simulink library "Vehicle_Outputs"  (R2025a)
settings: Solver=VariableStepAuto  StartTime=0.0  StopTime=10.0  RelTol=1e-3
libraries: $bdroot x30, Body_Utilities x12, sm_lib x4, nesl_utility x2
Description:
  | Simscape Vehicle Templates Library
  | 
  | Copyright 2018-2026 The MathWorks, Inc.
settings Model: Creator=smiller  LastModifiedBy=smiller
settings OptimizationCC: ReuseModelBlockBuffer=off
settings ModelReferenceCC: EnableRefExpFcnMdlSchedulingChecks=on
settings RTWCC: GPUComputeCapability=3.5

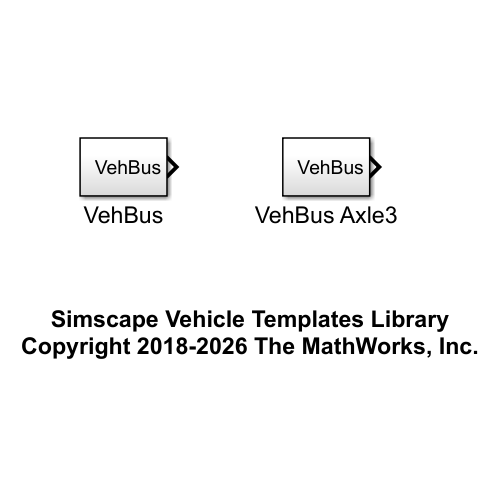
[thumbnail: Simulink's stored preview of the top-level diagram]
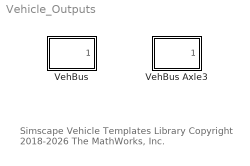
== system Vehicle_Outputs ==
  note: Simscape Vehicle Templates Library
      | Copyright 2018-2026 The MathWorks, Inc.
  VehBus : Subsystem
  VehBus Axle3 : Subsystem

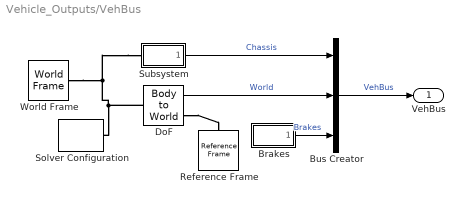
== system Vehicle_Outputs/VehBus ==
  Brakes : Subsystem
  Bus Creator : BusCreator  Inputs=3
  DoF : Body_Utilities/Body to World  VariantControl=Choice  LabelModeActiveChoice=Free  popup_BodyToWorld=Free  SpecifyPosTarget=on
  Reference Frame : sm_lib/Frames and Transforms/Reference Frame
  Solver Configuration : nesl_utility/Solver Configuration  PhysicalDomain=network_engine_domain  SubClassName=solver  LeftPortType=input  RightPortType=generic  Tones=[]  Harmonics=[]  SimulateNoise=off  Profile=off  UseLocalSampling=off  EnableSwitchedLinearOptims=on  FrequencyDomain=off  UseCCode=off  RelTol=0.001  AbsTol=1e-06  MinStep=1e-09  ToWorkspace=off  RevertToSquareIcSolve=off  NumHomotopyIterations=100  PhasorMode=off  PhasorModeNumHarmonics=1  ConsistencySolver=NEWTON_FTOL  IndexReductionMethod=DerivativeReplacement  DoDC=off  ResidualTolerance=1e-09  ConsistencyTolSource=GLOBAL  ConsistencyAbsTol=0.001  ConsistencyRelTol=0.001  ConsistencyTolFactor=0.001  UseLocalSolver=off  LocalSolverChoice=NE_BACKWARD_EULER_ADVANCER  ResolveIndetEquations=on  FunctionEvalNumThread=1  LocalSolverSampleTime=0.001  DoFixedCost=off  MaxNonlinIter=3  MaxModeIter=2  ComputeImpulses=off  ImpulseIterations=2  LinearAlgebra=auto  LinearAlgebraNumThread=0  EquationFormulation=NE_TIME_EF  DelaysMemoryBudget=1024  AutomaticFiltering=on  FilteringTimeConstant=0.001  PartitionStorageMethod=AS_NEEDED  PartitionMemoryBudget=1024  PartitionMethod=FAST  MultibodyUseLocalSolver=off  MultibodyLocalSolverChoice=ODE1  MultibodyLocalSolverSampleTime=0.001
  Subsystem : Subsystem
  World Frame : sm_lib/Frames and Transforms/World Frame
  VehBus : Outport  VectorParamsAs1DForOutWhenUnconnected=off
  wires:
  Bus Creator/1 -> VehBus/1  "VehBus"
  Subsystem/1(Chassis) -> Bus Creator/1  "Chassis"
  DoF/1 -> Bus Creator/2  "World"
  Brakes/1(Brakes) -> Bus Creator/3  "Brakes"
  connections:
  DoF/RConn1 -- Reference Frame/RConn1
  Subsystem/LConn1 -- Solver Configuration/RConn1 -- DoF/LConn1 -- World Frame/RConn1

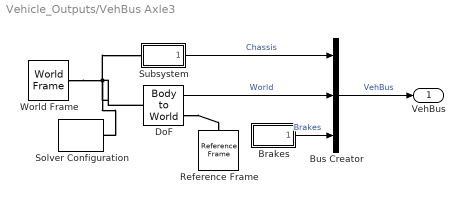
== system Vehicle_Outputs/VehBus Axle3 ==
  Brakes : Subsystem
  Bus Creator : BusCreator  Inputs=3
  DoF : Body_Utilities/Body to World  VariantControl=Choice  LabelModeActiveChoice=Free  popup_BodyToWorld=Free  SpecifyPosTarget=on
  Reference Frame : sm_lib/Frames and Transforms/Reference Frame
  Solver Configuration : nesl_utility/Solver Configuration  PhysicalDomain=network_engine_domain  SubClassName=solver  LeftPortType=input  RightPortType=generic  Tones=[]  Harmonics=[]  SimulateNoise=off  Profile=off  UseLocalSampling=off  EnableSwitchedLinearOptims=on  FrequencyDomain=off  UseCCode=off  RelTol=0.001  AbsTol=1e-06  MinStep=1e-09  ToWorkspace=off  RevertToSquareIcSolve=off  NumHomotopyIterations=100  PhasorMode=off  PhasorModeNumHarmonics=1  ConsistencySolver=NEWTON_FTOL  IndexReductionMethod=DerivativeReplacement  DoDC=off  ResidualTolerance=1e-09  ConsistencyTolSource=GLOBAL  ConsistencyAbsTol=0.001  ConsistencyRelTol=0.001  ConsistencyTolFactor=0.001  UseLocalSolver=off  LocalSolverChoice=NE_BACKWARD_EULER_ADVANCER  ResolveIndetEquations=on  FunctionEvalNumThread=1  LocalSolverSampleTime=0.001  DoFixedCost=off  MaxNonlinIter=3  MaxModeIter=2  ComputeImpulses=off  ImpulseIterations=2  LinearAlgebra=auto  LinearAlgebraNumThread=0  EquationFormulation=NE_TIME_EF  DelaysMemoryBudget=1024  AutomaticFiltering=on  FilteringTimeConstant=0.001  PartitionStorageMethod=AS_NEEDED  PartitionMemoryBudget=1024  PartitionMethod=FAST  MultibodyUseLocalSolver=off  MultibodyLocalSolverChoice=ODE1  MultibodyLocalSolverSampleTime=0.001
  Subsystem : Subsystem
  World Frame : sm_lib/Frames and Transforms/World Frame
  VehBus : Outport  VectorParamsAs1DForOutWhenUnconnected=off
  wires:
  Brakes/1(Brakes) -> Bus Creator/3  "Brakes"
  DoF/1 -> Bus Creator/2  "World"
  Subsystem/1(Chassis) -> Bus Creator/1  "Chassis"
  Bus Creator/1 -> VehBus/1  "VehBus"
  connections:
  World Frame/RConn1 -- DoF/LConn1 -- Solver Configuration/RConn1 -- Subsystem/LConn1
  DoF/RConn1 -- Reference Frame/RConn1

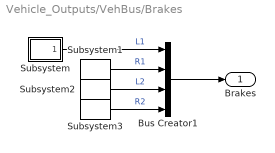
== system Vehicle_Outputs/VehBus/Brakes ==
  Bus Creator1 : BusCreator  Inputs=4
  Subsystem : Subsystem
  Subsystem1 : $bdroot/VehBus/Brakes/Subsystem  SystemSampleTime=-1  VariantActivationTime=update diagram  EmptyChoice=off  PassThrough=off  PassThroughVariantControl=(default)  EmptyChoiceVariantControl=(default)  AllowFlexibleInterface=on  Latency=0  AutoFrameSizeCalculation=off
  Subsystem2 : $bdroot/VehBus/Brakes/Subsystem  SystemSampleTime=-1  VariantActivationTime=update diagram  EmptyChoice=off  PassThrough=off  PassThroughVariantControl=(default)  EmptyChoiceVariantControl=(default)  AllowFlexibleInterface=on  Latency=0  AutoFrameSizeCalculation=off
  Subsystem3 : $bdroot/VehBus/Brakes/Subsystem  SystemSampleTime=-1  VariantActivationTime=update diagram  EmptyChoice=off  PassThrough=off  PassThroughVariantControl=(default)  EmptyChoiceVariantControl=(default)  AllowFlexibleInterface=on  Latency=0  AutoFrameSizeCalculation=off
  Brakes : Outport  VectorParamsAs1DForOutWhenUnconnected=off
  wires:
  Subsystem3/1 -> Bus Creator1/4  "R2"
  Subsystem2/1 -> Bus Creator1/3  "L2"
  Subsystem1/1 -> Bus Creator1/2  "R1"
  Subsystem/1(Whl) -> Bus Creator1/1  "L1"
  Bus Creator1/1 -> Brakes/1

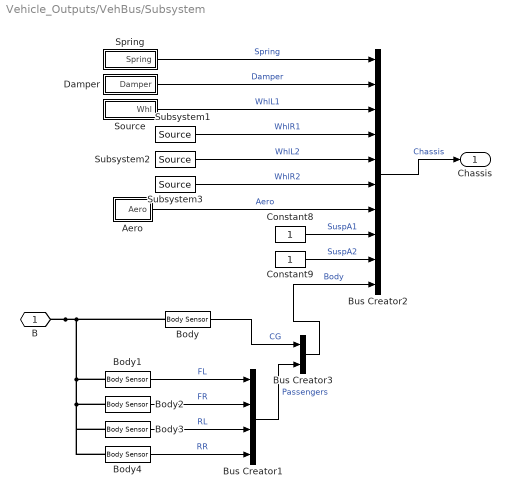
== system Vehicle_Outputs/VehBus/Subsystem ==
  Aero : Subsystem
  Body{,1..4} (5 alike) : Body_Utilities/Body Sensor  offset_body_sensor=Vehicle.Chassis.Body.sCG.Value
  Bus Creator1 : BusCreator  Inputs=4
  Bus Creator2 : BusCreator  Inputs=10
  Bus Creator3 : BusCreator  Inputs=2
  Constant8 : Constant
  Constant9 : Constant
  Damper : Subsystem
  Source : Subsystem
  Spring : Subsystem
  Subsystem1 : $bdroot/VehBus/Subsystem/Source  SystemSampleTime=-1  VariantActivationTime=update diagram  EmptyChoice=off  PassThrough=off  PassThroughVariantControl=(default)  EmptyChoiceVariantControl=(default)  AllowFlexibleInterface=on  Latency=0  AutoFrameSizeCalculation=off
  Subsystem2 : $bdroot/VehBus/Subsystem/Source  SystemSampleTime=-1  VariantActivationTime=update diagram  EmptyChoice=off  PassThrough=off  PassThroughVariantControl=(default)  EmptyChoiceVariantControl=(default)  AllowFlexibleInterface=on  Latency=0  AutoFrameSizeCalculation=off
  Subsystem3 : $bdroot/VehBus/Subsystem/Source  SystemSampleTime=-1  VariantActivationTime=update diagram  EmptyChoice=off  PassThrough=off  PassThroughVariantControl=(default)  EmptyChoiceVariantControl=(default)  AllowFlexibleInterface=on  Latency=0  AutoFrameSizeCalculation=off
  B : PMIOPort  Side=Left
  Chassis : Outport  VectorParamsAs1DForOutWhenUnconnected=off
  wires:
  Bus Creator1/1 -> Bus Creator3/2  "Passengers"
  Body4/1 -> Bus Creator1/4  "RR"
  Body3/1 -> Bus Creator1/3  "RL"
  Body2/1 -> Bus Creator1/2  "FR"
  Body1/1 -> Bus Creator1/1  "FL"
  Body/1 -> Bus Creator3/1  "CG"
  Bus Creator3/1 -> Bus Creator2/10  "Body"
  Aero/1(Aero) -> Bus Creator2/7  "Aero"
  Spring/1(Spring) -> Bus Creator2/1  "Spring"
  Source/1(Whl) -> Bus Creator2/3  "WhlL1"
  Constant9/1 -> Bus Creator2/9  "SuspA2"
  Constant8/1 -> Bus Creator2/8  "SuspA1"
  Subsystem3/1 -> Bus Creator2/6  "WhlR2"
  Subsystem2/1 -> Bus Creator2/5  "WhlL2"
  Bus Creator2/1 -> Chassis/1  "Chassis"
  Damper/1(Damper) -> Bus Creator2/2  "Damper"
  Subsystem1/1 -> Bus Creator2/4  "WhlR1"
  connections:
  B/RConn1 -- Body1/LConn1 -- Body2/LConn1 -- Body3/LConn1 -- Body4/LConn1 -- Body/LConn1

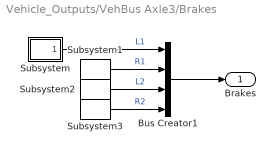
== system Vehicle_Outputs/VehBus Axle3/Brakes ==
  Bus Creator1 : BusCreator  Inputs=4
  Subsystem : Subsystem
  Subsystem1 : $bdroot/VehBus/Brakes/Subsystem  SystemSampleTime=-1  VariantActivationTime=update diagram  EmptyChoice=off  PassThrough=off  PassThroughVariantControl=(default)  EmptyChoiceVariantControl=(default)  AllowFlexibleInterface=on  Latency=0  AutoFrameSizeCalculation=off
  Subsystem2 : $bdroot/VehBus/Brakes/Subsystem  SystemSampleTime=-1  VariantActivationTime=update diagram  EmptyChoice=off  PassThrough=off  PassThroughVariantControl=(default)  EmptyChoiceVariantControl=(default)  AllowFlexibleInterface=on  Latency=0  AutoFrameSizeCalculation=off
  Subsystem3 : $bdroot/VehBus/Brakes/Subsystem  SystemSampleTime=-1  VariantActivationTime=update diagram  EmptyChoice=off  PassThrough=off  PassThroughVariantControl=(default)  EmptyChoiceVariantControl=(default)  AllowFlexibleInterface=on  Latency=0  AutoFrameSizeCalculation=off
  Brakes : Outport  VectorParamsAs1DForOutWhenUnconnected=off
  wires:
  Bus Creator1/1 -> Brakes/1
  Subsystem/1(Whl) -> Bus Creator1/1  "L1"
  Subsystem1/1 -> Bus Creator1/2  "R1"
  Subsystem2/1 -> Bus Creator1/3  "L2"
  Subsystem3/1 -> Bus Creator1/4  "R2"

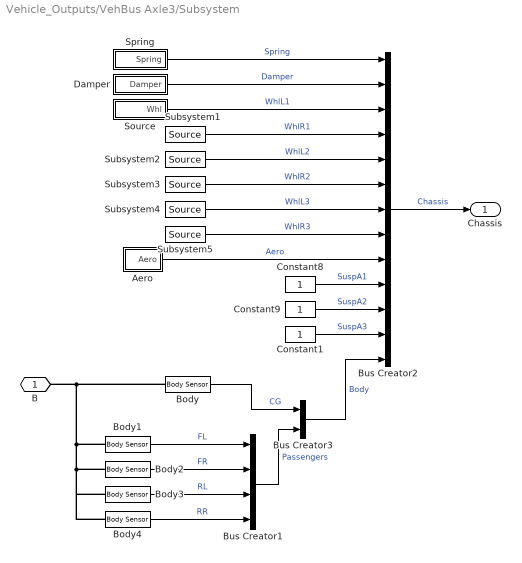
== system Vehicle_Outputs/VehBus Axle3/Subsystem ==
  Aero : Subsystem
  Body{,1..4} (5 alike) : Body_Utilities/Body Sensor  offset_body_sensor=Vehicle.Chassis.Body.sCG.Value
  Bus Creator1 : BusCreator  Inputs=4
  Bus Creator2 : BusCreator  Inputs=13
  Bus Creator3 : BusCreator  Inputs=2
  Constant1 : Constant
  Constant8 : Constant
  Constant9 : Constant
  Damper : Subsystem
  Source : Subsystem
  Spring : Subsystem
  Subsystem{1..5} (5 alike) : $bdroot/VehBus/Subsystem/Source  SystemSampleTime=-1  VariantActivationTime=update diagram  EmptyChoice=off  PassThrough=off  PassThroughVariantControl=(default)  EmptyChoiceVariantControl=(default)  AllowFlexibleInterface=on  Latency=0  AutoFrameSizeCalculation=off
  B : PMIOPort  Side=Left
  Chassis : Outport  VectorParamsAs1DForOutWhenUnconnected=off
  wires:
  Subsystem1/1 -> Bus Creator2/4  "WhlR1"
  Damper/1(Damper) -> Bus Creator2/2  "Damper"
  Bus Creator2/1 -> Chassis/1  "Chassis"
  Subsystem2/1 -> Bus Creator2/5  "WhlL2"
  Subsystem3/1 -> Bus Creator2/6  "WhlR2"
  Constant8/1 -> Bus Creator2/10  "SuspA1"
  Constant9/1 -> Bus Creator2/11  "SuspA2"
  Source/1(Whl) -> Bus Creator2/3  "WhlL1"
  Spring/1(Spring) -> Bus Creator2/1  "Spring"
  Aero/1(Aero) -> Bus Creator2/9  "Aero"
  Bus Creator3/1 -> Bus Creator2/13  "Body"
  Body/1 -> Bus Creator3/1  "CG"
  Body1/1 -> Bus Creator1/1  "FL"
  Body2/1 -> Bus Creator1/2  "FR"
  Body3/1 -> Bus Creator1/3  "RL"
  Body4/1 -> Bus Creator1/4  "RR"
  Bus Creator1/1 -> Bus Creator3/2  "Passengers"
  Subsystem5/1 -> Bus Creator2/8  "WhlR3"
  Subsystem4/1 -> Bus Creator2/7  "WhlL3"
  Constant1/1 -> Bus Creator2/12  "SuspA3"
  connections:
  Body/LConn1 -- Body4/LConn1 -- Body3/LConn1 -- Body2/LConn1 -- Body1/LConn1 -- B/RConn1

== system Vehicle_Outputs/VehBus/Brakes/Subsystem ==
  Bus Creator : BusCreator  Inputs=2
  Constant : Constant
  Constant1 : Constant
  Whl : Outport  VectorParamsAs1DForOutWhenUnconnected=off
  wires:
  Constant1/1 -> Bus Creator/2  "p"
  Bus Creator/1 -> Whl/1
  Constant/1 -> Bus Creator/1  "trq"

== system Vehicle_Outputs/VehBus/Subsystem/Aero ==
  Bus Creator : BusCreator  Inputs=2
  Constant1 : Constant
  Constant3 : Constant
  Aero : Outport  VectorParamsAs1DForOutWhenUnconnected=off
  wires:
  Bus Creator/1 -> Aero/1  "Aero"
  Constant1/1 -> Bus Creator/2  "Fz"
  Constant3/1 -> Bus Creator/1  "Fx"

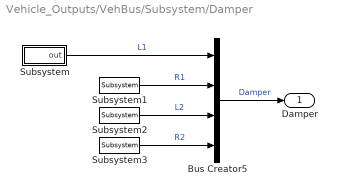
== system Vehicle_Outputs/VehBus/Subsystem/Damper ==
  Bus Creator5 : BusCreator  Inputs=4
  Subsystem : Subsystem
  Subsystem1 : $bdroot/VehBus/Subsystem/Damper/Subsystem  SystemSampleTime=-1  VariantActivationTime=update diagram  EmptyChoice=off  PassThrough=off  PassThroughVariantControl=(default)  EmptyChoiceVariantControl=(default)  AllowFlexibleInterface=on  Latency=0  AutoFrameSizeCalculation=off
  Subsystem2 : $bdroot/VehBus/Subsystem/Damper/Subsystem  SystemSampleTime=-1  VariantActivationTime=update diagram  EmptyChoice=off  PassThrough=off  PassThroughVariantControl=(default)  EmptyChoiceVariantControl=(default)  AllowFlexibleInterface=on  Latency=0  AutoFrameSizeCalculation=off
  Subsystem3 : $bdroot/VehBus/Subsystem/Damper/Subsystem  SystemSampleTime=-1  VariantActivationTime=update diagram  EmptyChoice=off  PassThrough=off  PassThroughVariantControl=(default)  EmptyChoiceVariantControl=(default)  AllowFlexibleInterface=on  Latency=0  AutoFrameSizeCalculation=off
  Damper : Outport  VectorParamsAs1DForOutWhenUnconnected=off
  wires:
  Subsystem/1(out) -> Bus Creator5/1  "L1"
  Subsystem2/1 -> Bus Creator5/3  "L2"
  Bus Creator5/1 -> Damper/1  "Damper"
  Subsystem1/1 -> Bus Creator5/2  "R1"
  Subsystem3/1 -> Bus Creator5/4  "R2"

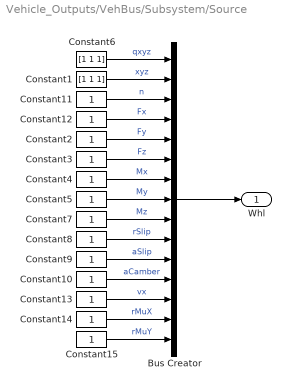
== system Vehicle_Outputs/VehBus/Subsystem/Source ==
  Bus Creator : BusCreator  Inputs=15
  Constant1 : Constant  Value=[1 1 1]
  Constant{2..5,7..15} (13 alike) : Constant
  Constant6 : Constant  Value=[1 1 1]
  Whl : Outport  VectorParamsAs1DForOutWhenUnconnected=off
  wires:
  Constant15/1 -> Bus Creator/15  "rMuY"
  Constant14/1 -> Bus Creator/14  "rMuX"
  Constant13/1 -> Bus Creator/13  "vx"
  Constant10/1 -> Bus Creator/12  "aCamber"
  Constant9/1 -> Bus Creator/11  "aSlip"
  Constant8/1 -> Bus Creator/10  "rSlip"
  Constant7/1 -> Bus Creator/9  "Mz"
  Constant5/1 -> Bus Creator/8  "My"
  Constant4/1 -> Bus Creator/7  "Mx"
  Constant3/1 -> Bus Creator/6  "Fz"
  Constant2/1 -> Bus Creator/5  "Fy"
  Bus Creator/1 -> Whl/1
  Constant6/1 -> Bus Creator/1  "qxyz"
  Constant1/1 -> Bus Creator/2  "xyz"
  Constant12/1 -> Bus Creator/4  "Fx"
  Constant11/1 -> Bus Creator/3  "n"

== system Vehicle_Outputs/VehBus/Subsystem/Spring ==
  Bus Creator5 : BusCreator  Inputs=4
  Source : Subsystem
  Source1 : $bdroot/VehBus/Subsystem/Spring/Source  SystemSampleTime=-1  VariantActivationTime=update diagram  EmptyChoice=off  PassThrough=off  PassThroughVariantControl=(default)  EmptyChoiceVariantControl=(default)  AllowFlexibleInterface=on  Latency=0  AutoFrameSizeCalculation=off
  Source2 : $bdroot/VehBus/Subsystem/Spring/Source  SystemSampleTime=-1  VariantActivationTime=update diagram  EmptyChoice=off  PassThrough=off  PassThroughVariantControl=(default)  EmptyChoiceVariantControl=(default)  AllowFlexibleInterface=on  Latency=0  AutoFrameSizeCalculation=off
  Source3 : $bdroot/VehBus/Subsystem/Spring/Source  SystemSampleTime=-1  VariantActivationTime=update diagram  EmptyChoice=off  PassThrough=off  PassThroughVariantControl=(default)  EmptyChoiceVariantControl=(default)  AllowFlexibleInterface=on  Latency=0  AutoFrameSizeCalculation=off
  Spring : Outport  VectorParamsAs1DForOutWhenUnconnected=off
  wires:
  Source/1(out) -> Bus Creator5/1  "L1"
  Source3/1 -> Bus Creator5/4  "R2"
  Source2/1 -> Bus Creator5/3  "L2"
  Source1/1 -> Bus Creator5/2  "R1"
  Bus Creator5/1 -> Spring/1  "Spring"

== system Vehicle_Outputs/VehBus Axle3/Brakes/Subsystem ==
  Bus Creator : BusCreator  Inputs=2
  Constant : Constant
  Constant1 : Constant
  Whl : Outport  VectorParamsAs1DForOutWhenUnconnected=off
  wires:
  Constant/1 -> Bus Creator/1  "trq"
  Bus Creator/1 -> Whl/1
  Constant1/1 -> Bus Creator/2  "p"

== system Vehicle_Outputs/VehBus Axle3/Subsystem/Aero ==
  Bus Creator : BusCreator  Inputs=2
  Constant1 : Constant
  Constant3 : Constant
  Aero : Outport  VectorParamsAs1DForOutWhenUnconnected=off
  wires:
  Constant3/1 -> Bus Creator/1  "Fx"
  Constant1/1 -> Bus Creator/2  "Fz"
  Bus Creator/1 -> Aero/1  "Aero"

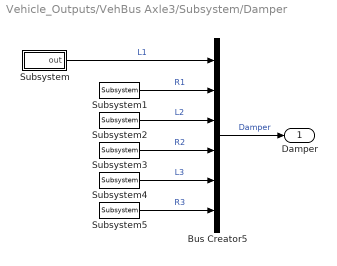
== system Vehicle_Outputs/VehBus Axle3/Subsystem/Damper ==
  Bus Creator5 : BusCreator  Inputs=6
  Subsystem : Subsystem
  Subsystem{1..5} (5 alike) : $bdroot/VehBus/Subsystem/Damper/Subsystem  SystemSampleTime=-1  VariantActivationTime=update diagram  EmptyChoice=off  PassThrough=off  PassThroughVariantControl=(default)  EmptyChoiceVariantControl=(default)  AllowFlexibleInterface=on  Latency=0  AutoFrameSizeCalculation=off
  Damper : Outport  VectorParamsAs1DForOutWhenUnconnected=off
  wires:
  Subsystem3/1 -> Bus Creator5/4  "R2"
  Subsystem1/1 -> Bus Creator5/2  "R1"
  Bus Creator5/1 -> Damper/1  "Damper"
  Subsystem2/1 -> Bus Creator5/3  "L2"
  Subsystem/1(out) -> Bus Creator5/1  "L1"
  Subsystem4/1 -> Bus Creator5/5  "L3"
  Subsystem5/1 -> Bus Creator5/6  "R3"

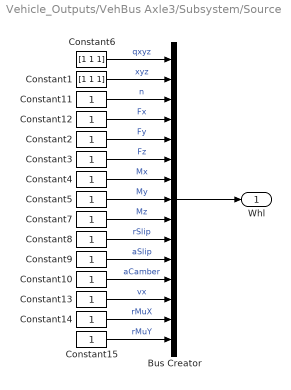
== system Vehicle_Outputs/VehBus Axle3/Subsystem/Source ==
  Bus Creator : BusCreator  Inputs=15
  Constant1 : Constant  Value=[1 1 1]
  Constant{2..5,7..15} (13 alike) : Constant
  Constant6 : Constant  Value=[1 1 1]
  Whl : Outport  VectorParamsAs1DForOutWhenUnconnected=off
  wires:
  Constant11/1 -> Bus Creator/3  "n"
  Constant12/1 -> Bus Creator/4  "Fx"
  Constant1/1 -> Bus Creator/2  "xyz"
  Constant6/1 -> Bus Creator/1  "qxyz"
  Bus Creator/1 -> Whl/1
  Constant2/1 -> Bus Creator/5  "Fy"
  Constant3/1 -> Bus Creator/6  "Fz"
  Constant4/1 -> Bus Creator/7  "Mx"
  Constant5/1 -> Bus Creator/8  "My"
  Constant7/1 -> Bus Creator/9  "Mz"
  Constant8/1 -> Bus Creator/10  "rSlip"
  Constant9/1 -> Bus Creator/11  "aSlip"
  Constant10/1 -> Bus Creator/12  "aCamber"
  Constant13/1 -> Bus Creator/13  "vx"
  Constant14/1 -> Bus Creator/14  "rMuX"
  Constant15/1 -> Bus Creator/15  "rMuY"

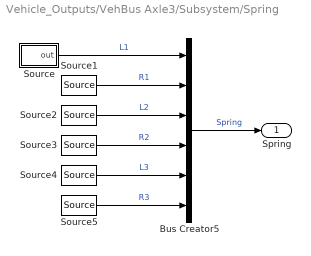
== system Vehicle_Outputs/VehBus Axle3/Subsystem/Spring ==
  Bus Creator5 : BusCreator  Inputs=6
  Source : Subsystem
  Source{1..5} (5 alike) : $bdroot/VehBus/Subsystem/Spring/Source  SystemSampleTime=-1  VariantActivationTime=update diagram  EmptyChoice=off  PassThrough=off  PassThroughVariantControl=(default)  EmptyChoiceVariantControl=(default)  AllowFlexibleInterface=on  Latency=0  AutoFrameSizeCalculation=off
  Spring : Outport  VectorParamsAs1DForOutWhenUnconnected=off
  wires:
  Bus Creator5/1 -> Spring/1  "Spring"
  Source1/1 -> Bus Creator5/2  "R1"
  Source2/1 -> Bus Creator5/3  "L2"
  Source3/1 -> Bus Creator5/4  "R2"
  Source/1(out) -> Bus Creator5/1  "L1"
  Source5/1 -> Bus Creator5/6  "R3"
  Source4/1 -> Bus Creator5/5  "L3"

== system Vehicle_Outputs/VehBus/Subsystem/Damper/Subsystem ==
  Bus Creator : BusCreator  Inputs=4
  Constant{1..4} (4 alike) : Constant
  out : Outport  VectorParamsAs1DForOutWhenUnconnected=off
  wires:
  Constant4/1 -> Bus Creator/1  "FDamper"
  Constant1/1 -> Bus Creator/2  "FBumpstop"
  Constant3/1 -> Bus Creator/4  "vDamper"
  Bus Creator/1 -> out/1
  Constant2/1 -> Bus Creator/3  "xDamper"

== system Vehicle_Outputs/VehBus/Subsystem/Spring/Source ==
  Bus Creator : BusCreator  Inputs=2
  Constant1 : Constant
  Constant4 : Constant
  out : Outport  VectorParamsAs1DForOutWhenUnconnected=off
  wires:
  Bus Creator/1 -> out/1
  Constant4/1 -> Bus Creator/1  "xSpring"
  Constant1/1 -> Bus Creator/2  "FSpring"

== system Vehicle_Outputs/VehBus Axle3/Subsystem/Damper/Subsystem ==
  Bus Creator : BusCreator  Inputs=4
  Constant{1..4} (4 alike) : Constant
  out : Outport  VectorParamsAs1DForOutWhenUnconnected=off
  wires:
  Constant2/1 -> Bus Creator/3  "xDamper"
  Bus Creator/1 -> out/1
  Constant3/1 -> Bus Creator/4  "vDamper"
  Constant1/1 -> Bus Creator/2  "FBumpstop"
  Constant4/1 -> Bus Creator/1  "FDamper"

== system Vehicle_Outputs/VehBus Axle3/Subsystem/Spring/Source ==
  Bus Creator : BusCreator  Inputs=2
  Constant1 : Constant
  Constant4 : Constant
  out : Outport  VectorParamsAs1DForOutWhenUnconnected=off
  wires:
  Constant1/1 -> Bus Creator/2  "FSpring"
  Constant4/1 -> Bus Creator/1  "xSpring"
  Bus Creator/1 -> out/1
